simulink model "MassSpringDamper_Oct9_Simulink"  (R2026b)
settings: Solver=VariableStepAuto
libraries: fl_lib x14, nesl_utility x7
settings Model: Creator=Alan  LastModifiedBy=Alan
settings SimscapeCC: SimscapeLogType=all  SimscapeNominalValues="[{\"value\":\"1\",\"unit\":\"A\"},{\"value\":\"1\",\"unit\":\"bar\"},{\"value\":\"1\",\"unit\":\"cm^2\"},{\"value\":\"1\",\"unit\":\"cm^3/s\"},{\"value\":\"1\",\"unit\":\"kJ/kg\"},{\"value\":\"1\",\"unit\":\"kW\"},{\"value\":\"1\",\"unit\":\"l\"},{\"value\":\"1\",\"unit\":\"N\"},{\"value\":\"1\",\"unit\":\"N*m\"},{\"value\":\"1\",\"unit\":\"V\"},{\"value\":\"0.001\",\"unit\":\"Wb\"}]"  SimscapeUseEnergyAccounting=off

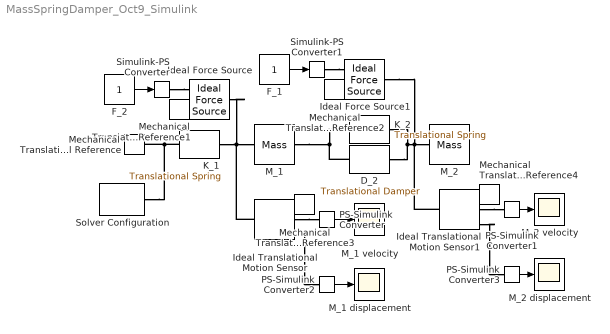
== system MassSpringDamper_Oct9_Simulink ==
  D_2 : fl_lib/Mechanical/Translational Elements/Translational Damper  D=100 N*s/m  v_specify=off  v_priority=None  v=0 m/s  v_nominal_specify=off  v_nominal_value=1  v_nominal_unit=m/s  f_specify=off  f_priority=None  f=0 N  f_nominal_specify=off  f_nominal_value=1  f_nominal_unit=N
  F_1 : Constant
  F_2 : Constant
  Ideal Force Source : fl_lib/Mechanical/Mechanical Sources/Ideal Force Source
  Ideal Force Source1 : fl_lib/Mechanical/Mechanical Sources/Ideal Force Source
  Ideal Translational Motion Sensor : fl_lib/Mechanical/Mechanical Sensors/Ideal Translational Motion Sensor  reference=foundation.enum.MeasurementReference.difference  acceleration_port=false  velocity_port=true  position_port=true  offset=0 m
  Ideal Translational Motion Sensor1 : fl_lib/Mechanical/Mechanical Sensors/Ideal Translational Motion Sensor  reference=foundation.enum.MeasurementReference.difference  acceleration_port=false  velocity_port=true  position_port=true  offset=0 m
  K_1 : fl_lib/Mechanical/Translational Elements/Translational Spring  spr_rate=1000 N/m  v_specify=off  v_priority=None  v=0 m/s  v_nominal_specify=off  v_nominal_value=1  v_nominal_unit=m/s  f_specify=off  f_priority=None  f=0 N  f_nominal_specify=off  f_nominal_value=1  f_nominal_unit=N  x_specify=off  x_priority=High  x=0 m  x_nominal_specify=off  x_nominal_value=1  x_nominal_unit=m
  K_2 : fl_lib/Mechanical/Translational Elements/Translational Spring  spr_rate=1000 N/m  v_specify=off  v_priority=None  v=0 m/s  v_nominal_specify=off  v_nominal_value=1  v_nominal_unit=m/s  f_specify=off  f_priority=None  f=0 N  f_nominal_specify=off  f_nominal_value=1  f_nominal_unit=N  x_specify=off  x_priority=High  x=0 m  x_nominal_specify=off  x_nominal_value=1  x_nominal_unit=m
  M_1 : fl_lib/Mechanical/Translational Elements/Mass  mass=1 kg  num_ports=foundation.enum.numPorts2.two  v_specify=off  v_priority=High  v=0 m/s  v_nominal_specify=off  v_nominal_value=1  v_nominal_unit=m/s  f_specify=off  f_priority=None  f=0 N  f_nominal_specify=off  f_nominal_value=1  f_nominal_unit=N
  M_1 displacement : Scope
      settings: Title=Displacement of M_1 vs Time  ActiveDisplayYMinimum=-0.00047441515055755276  ActiveDisplayYMaximum=0.0042697363550179756  YLabel=Displacement  DataLoggingVariableName=ScopeData2
  M_1 velocity : Scope
      settings: Title=Velocity of M_1 vs Time  ActiveDisplayYMinimum=-0.045593641125860229  ActiveDisplayYMaximum=0.051469672148032886  YLabel=Velocity
  M_2 : fl_lib/Mechanical/Translational Elements/Mass  mass=1 kg  num_ports=foundation.enum.numPorts2.one  v_specify=off  v_priority=High  v=0 m/s  v_nominal_specify=off  v_nominal_value=1  v_nominal_unit=m/s  f_specify=off  f_priority=None  f=0 N  f_nominal_specify=off  f_nominal_value=1  f_nominal_unit=N
  M_2 displacement : Scope
      settings: Title=Displacement of M_2 vs Time  ActiveDisplayYMinimum=-0.00059223611289947438  ActiveDisplayYMaximum=0.0053301250160952707  YLabel=Displacement  DataLoggingVariableName=ScopeData3
  M_2 velocity : Scope
      settings: Title=Velocity of M_2 vs Time  ActiveDisplayYMinimum=-0.0487810496706024  ActiveDisplayYMaximum=0.060110966258236739  YLabel=Velocity
  Mechanical Translational Reference{,1..4} (5 alike) : fl_lib/Mechanical/Translational Elements/Mechanical Translational Reference
  PS-Simulink Converter{,1..3} (4 alike) : nesl_utility/PS-Simulink Converter  PhysicalDomain=network_engine_domain  SubClassName=ps_output  LeftPortType=input  RightPortType=output  PseudoPeriodic=off  Frequencies=[]  VectorFormat=inherit  Unit=inherit  AffineConversion=off
  Simulink-PS Converter : nesl_utility/Simulink-PS Converter  PhysicalDomain=network_engine_domain  SubClassName=ps_input  LeftPortType=input  RightPortType=output  PseudoPeriodic=off  Frequencies=[]  NoiseDistribution=none  NoiseParameters=[]  Unit=1  AffineConversion=off  FilteringAndDerivatives=provide  SimscapeFilterOrder=1  InputFilterTimeConstant=0.001  UdotUserProvided=0
  Simulink-PS Converter1 : nesl_utility/Simulink-PS Converter  PhysicalDomain=network_engine_domain  SubClassName=ps_input  LeftPortType=input  RightPortType=output  PseudoPeriodic=off  Frequencies=[]  NoiseDistribution=none  NoiseParameters=[]  Unit=1  AffineConversion=off  FilteringAndDerivatives=provide  SimscapeFilterOrder=1  InputFilterTimeConstant=0.001  UdotUserProvided=0
  Solver Configuration : nesl_utility/Solver Configuration  PhysicalDomain=network_engine_domain  SubClassName=solver  LeftPortType=input  RightPortType=generic  Tones=[]  Harmonics=[]  SimulateNoise=off  Profile=off  UseLocalSampling=off  EnableSwitchedLinearOptims=on  FrequencyDomain=off  UseCCode=off  RelTol=0.001  AbsTol=0.001  MinStep=1e-09  ToWorkspace=off  RevertToSquareIcSolve=off  NumHomotopyIterations=100  PhasorMode=off  PhasorModeNumHarmonics=1  ConsistencySolver=NEWTON_XTOL_AFTER_FTOL  CanonicalOrdering=CANONICAL  OptimizeIntermediates=OPTIMIZED  MulticoreSolverChoice=BACKWARD_EULER  IndexReductionMethod=DerivativeReplacement  DoDC=off  ResidualTolerance=1e-09  ConsistencyTolSource=GLOBAL  ConsistencyAbsTol=0.001  ConsistencyRelTol=0.001  ConsistencyTolFactor=0.001  UseLocalSolver=off  LocalSolverChoice=NE_BACKWARD_EULER_ADVANCER  ResolveIndetEquations=on  FunctionEvalNumThread=1  LocalSolverSampleTime=0.001  DoFixedCost=off  MaxNonlinIter=3  MaxModeIter=2  ComputeImpulses=off  ImpulseIterations=2  LinearAlgebra=auto  LinearAlgebraNumThread=0  EquationFormulation=NE_TIME_EF  DelaysMemoryBudget=1024  AutomaticFiltering=on  FilteringTimeConstant=0.001  PartitionStorageMethod=AS_NEEDED  PartitionMemoryBudget=1024  PartitionMethod=BALANCED  MultibodyUseLocalSolver=off  MultibodyLocalSolverChoice=ODE1  MultibodyLocalSolverSampleTime=0.001
  wires:
  F_2/1 -> Simulink-PS Converter/1
  F_1/1 -> Simulink-PS Converter1/1
  PS-Simulink Converter/1 -> M_1 velocity/1
  PS-Simulink Converter1/1 -> M_2 velocity/1
  PS-Simulink Converter2/1 -> M_1 displacement/1
  PS-Simulink Converter3/1 -> M_2 displacement/1
  connections:
  K_1/LConn1 -- Solver Configuration/RConn1 -- Mechanical Translational Reference/LConn1
  K_1/RConn1 -- Ideal Translational Motion Sensor/LConn1 -- Ideal Force Source/LConn1 -- M_1/RConn1
  M_1/LConn1 -- K_2/LConn1 -- D_2/LConn1
  Mechanical Translational Reference1/LConn1 -- Ideal Force Source/RConn2
  Mechanical Translational Reference2/LConn1 -- Ideal Force Source1/RConn2
  K_2/RConn1 -- D_2/RConn1 -- Ideal Force Source1/LConn1 -- Ideal Translational Motion Sensor1/LConn1 -- M_2/LConn1
  Simulink-PS Converter/RConn1 -- Ideal Force Source/RConn1
  Simulink-PS Converter1/RConn1 -- Ideal Force Source1/RConn1
  Mechanical Translational Reference3/LConn1 -- Ideal Translational Motion Sensor/RConn1
  Mechanical Translational Reference4/LConn1 -- Ideal Translational Motion Sensor1/RConn1
  Ideal Translational Motion Sensor/RConn2 -- PS-Simulink Converter/LConn1
  Ideal Translational Motion Sensor1/RConn2 -- PS-Simulink Converter1/LConn1
  Ideal Translational Motion Sensor/RConn3 -- PS-Simulink Converter2/LConn1
  Ideal Translational Motion Sensor1/RConn3 -- PS-Simulink Converter3/LConn1
